simulink model "test_LQI_x"  (R2025b)
settings: Solver=VariableStepAuto  StartTime=0.0  StopTime=15  RelTol=1e-3
values from neighbouring files (symbols this model uses):
  Kd = 0.8 * K_aug(2)    [gains_LQI.m]
  Kd_theta = K_aug_theta(2)    [gains_LQI.m]
  Kd_x = 0.28    [gains_LQI.m]
  Ki = 0.8 * K_aug(3)    [gains_LQI.m]
  Ki_theta = K_aug_theta(3)    [gains_LQI.m]
  Kp = 0.8 * K_aug(1)    [gains_LQI.m]
  Kp_theta = K_aug_theta(1)    [gains_LQI.m]
  Kp_x = 0.23    [gains_LQI.m]
  tau = 1.2    [gains_LQI.m]
undefined symbols (not defined in the file or in its folder): DiscIntNeverNeededParam
libraries: simulink x2
settings Model: Creator=anoua  LastModifiedBy=anoua

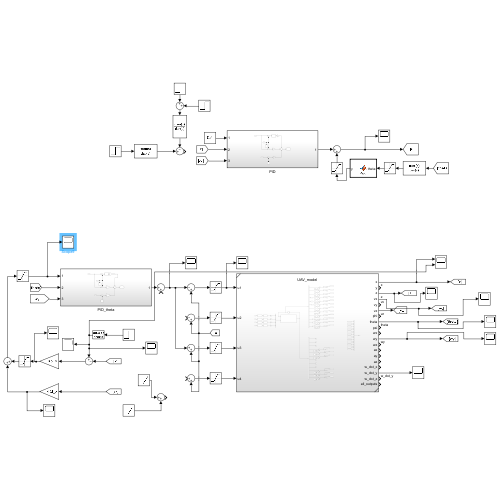
[thumbnail: Simulink's stored preview of the top-level diagram]
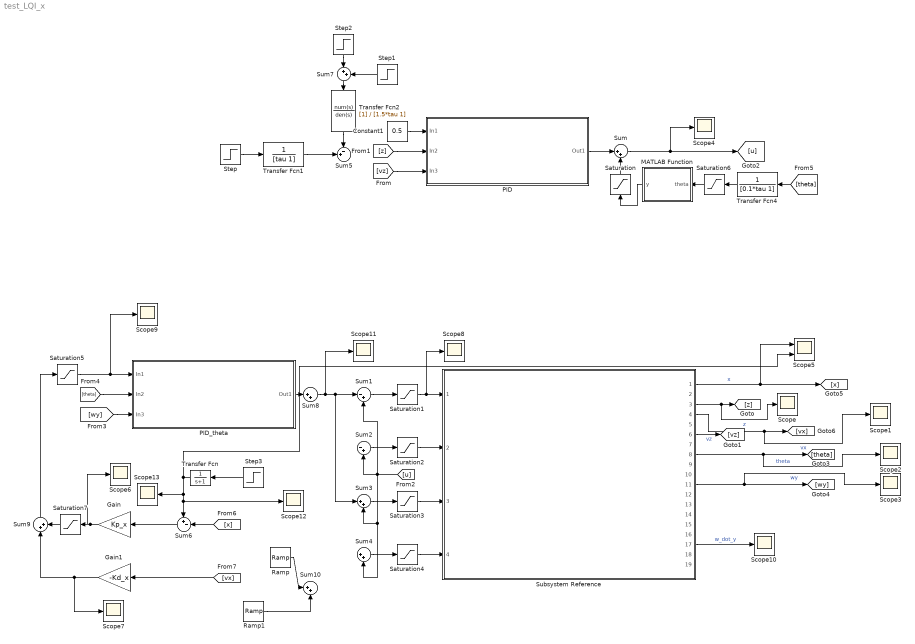
== system test_LQI_x ==
  Constant1 : Constant  Value=0.5
  Gain : Gain  Gain=Kp_x
  Gain1 : Gain  Gain=-Kd_x
  MATLAB Function : MATLAB Function  TreatAsAtomicUnit=on
  PID : Subsystem
  PID_theta : Subsystem
  Ramp : simulink/Sources/Ramp  slope=2  start=4  InitialOutput=0
  Ramp1 : simulink/Sources/Ramp  slope=-2  start=10  InitialOutput=0
  Saturation : Saturate  LowerLimit=0.3
  Saturation{1..4} (4 alike) : Saturate  UpperLimit=1  LowerLimit=-1
  Saturation5 : Saturate  UpperLimit=0.3  LowerLimit=-0.3  LinearizeAsGain=off
  Saturation6 : Saturate  UpperLimit=0.1  LowerLimit=0.1
  Saturation7 : Saturate  UpperLimit=1.5  LowerLimit=-1.5
  Scope{,1..4,6..13} (13 alike) : Scope
      Scope settings: ActiveDisplayYMinimum=-0.14718126227683057  ActiveDisplayYMaximum=0.70256454123979917
      Scope1 settings: ActiveDisplayYMinimum=-0.689477140233383  ActiveDisplayYMaximum=6.1817348155800982
      Scope10 settings: ActiveDisplayYMinimum=-8.1395929845312978  ActiveDisplayYMaximum=7.926459001284055  DataLoggingVariableName=ScopeData11
      Scope11 settings: ActiveDisplayYMinimum=-0.092583056017124382  ActiveDisplayYMaximum=0.10885517876194711  DataLoggingVariableName=ScopeData12
      Scope12 settings: ActiveDisplayYMinimum=-0.2209054413815989  ActiveDisplayYMaximum=0.24676727126462211  DataLoggingVariableName=ScopeData13
      Scope13 settings: ActiveDisplayYMinimum=-12.499998593310311  ActiveDisplayYMaximum=112.49998733979282  DataLoggingVariableName=ScopeData14
      Scope2 settings: ActiveDisplayYMinimum=-0.2429354271452315  ActiveDisplayYMaximum=0.30371803147303827  DataLoggingVariableName=ScopeData2
      Scope3 settings: ActiveDisplayYMinimum=-0.35804331506939135  ActiveDisplayYMaximum=2.2543304965066233  DataLoggingVariableName=ScopeData5
      Scope4 settings: ActiveDisplayYMinimum=-4.4218137268268194  ActiveDisplayYMaximum=39.350730126019634  DataLoggingVariableName=ScopeData4
      Scope6 settings: ActiveDisplayYMinimum=-3.5759205292689886  ActiveDisplayYMaximum=0.41468962885277622  DataLoggingVariableName=ScopeData7
      Scope7 settings: ActiveDisplayYMinimum=-1.5368936479557955  ActiveDisplayYMaximum=0.17077884596504492  DataLoggingVariableName=ScopeData8
      Scope8 settings: ActiveDisplayYMinimum=-0.17670639288242362  ActiveDisplayYMaximum=1.1307451547647138  DataLoggingVariableName=ScopeData9
      Scope9 settings: ActiveDisplayYMinimum=-0.28830610505236332  ActiveDisplayYMaximum=0.27997211142053136  DataLoggingVariableName=ScopeData10
  Scope5 : Scope  NumInputPorts=2
      settings: ActiveDisplayYMinimum=-0.6266529637915077  ActiveDisplayYMaximum=5.6296559852329642  DataLoggingVariableName=ScopeData6
  Step : Step  Time=0  After=0.5  SampleTime=0
  Step1 : Step  Time=16  After=0.70  SampleTime=0
  Step2 : Step  Time=22  After=0.05  SampleTime=0
  Step3 : Step  Time=4  After=5  SampleTime=0
  Subsystem Reference : Subsystem  ReferencedSubsystem=UAV_model
  Sum{,3..4,7..10} (7 alike) : Sum  Inputs=|++
  Sum1 : Sum  Inputs=|-+
  Sum2 : Sum  Inputs=|-+
  Sum5 : Sum  Inputs=-+|
  Sum6 : Sum  Inputs=+-|
  Transfer Fcn : TransferFcn  Denominator=[1 1]
  Transfer Fcn1 : TransferFcn  Denominator=[tau 1]
  Transfer Fcn2 : TransferFcn  Denominator=[1.5*tau 1]
  Transfer Fcn4 : TransferFcn  Denominator=[0.1*tau 1]
  wires:
  Subsystem Reference/3 -> Scope/1, [z]  "z"
  Sum/1 -> [u], Scope4/1
  [z] -> PID/2(In2)
  PID/1(Out1) -> Sum/1
  [vz] -> PID/3(In3)
  Sum2/1 -> Saturation2/1
  Sum7/1 -> Transfer Fcn2/1
  [u] -> Sum4/2, Sum3/2, Sum1/2, Sum2/2
  Saturation4/1 -> Subsystem Reference/4
  [theta] -> PID_theta/2(In2)
  Step1/1 -> Sum7/2
  [wy] -> PID_theta/3(In3)
  Step2/1 -> Sum7/1
  Transfer Fcn2/1 -> Sum5/1
  Saturation1/1 -> Scope8/1, Subsystem Reference/1
  Transfer Fcn1/1 -> Sum5/2
  Sum3/1 -> Saturation3/1
  Saturation3/1 -> Subsystem Reference/3
  Sum4/1 -> Saturation4/1
  Step/1 -> Transfer Fcn1/1
  Saturation2/1 -> Subsystem Reference/2
  Sum1/1 -> Saturation1/1
  Sum8/1 -> Scope11/1, Sum3/1, Sum1/1
  Subsystem Reference/11 -> Scope3/1, [wy]  "wy"
  Subsystem Reference/1 -> Scope5/1, [x]  "x"
  Constant1/1 -> PID/1(In1)
  MATLAB Function/1(y) -> Saturation/1
  [theta] -> Transfer Fcn4/1
  Transfer Fcn4/1 -> Saturation6/1
  Saturation/1 -> Sum/2
  Subsystem Reference/8 -> Scope2/1, [theta]  "theta"
  Subsystem Reference/17 -> Scope10/1  "w_dot_y"
  PID_theta/1(Out1) -> Sum8/1
  Subsystem Reference/4 -> Scope1/1, [vx]  "vx"
  [x] -> Sum6/2
  Sum6/1 -> Gain/1
  [vx] -> Gain1/1
  Gain/1 -> Scope6/1, Saturation7/1
  Gain1/1 -> Sum9/1, Scope7/1
  Sum9/1 -> Saturation5/1
  Saturation6/1 -> MATLAB Function/1(theta)
  Subsystem Reference/6 -> [vz]  "vz"
  Saturation5/1 -> Scope9/1, PID_theta/1(In1)
  Transfer Fcn/1 -> Scope13/1, Scope12/1, Sum6/1, Scope5/2
  Ramp/1 -> Sum10/1
  Ramp1/1 -> Sum10/2
  Step3/1 -> Transfer Fcn/1
  Saturation7/1 -> Sum9/2

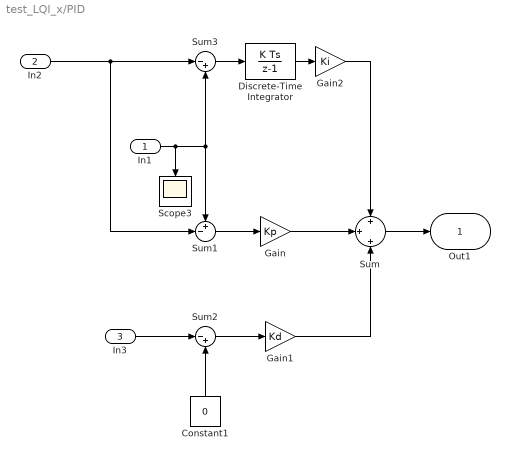
== system test_LQI_x/PID ==
  In1 : Inport
  In2 : Inport  Port=2
  In3 : Inport  Port=3
  Constant1 : Constant  Value=0
  Discrete-Time Integrator : DiscreteIntegrator  SampleTime=-1  LimitOutput=on  UpperSaturationLimit=1/Ki  LowerSaturationLimit=-1/Ki  ICPrevOutput=DiscIntNeverNeededParam  ICPrevScaledInput=DiscIntNeverNeededParam
  Gain : Gain  Gain=Kp
  Gain1 : Gain  Gain=Kd
  Gain2 : Gain  Gain=Ki
  Scope3 : Scope
      settings: ActiveDisplayYMinimum=-0.53484809981403014  ActiveDisplayYMaximum=1.6271171549271228  DataLoggingVariableName=ScopeData3
  Sum : Sum  Inputs=+|+|+
  Sum1 : Sum  Inputs=+-|
  Sum2 : Sum  Inputs=|-+
  Sum3 : Sum  Inputs=|-+
  Out1 : Outport
  wires:
  Gain2/1 -> Sum/1
  Gain/1 -> Sum/2
  Sum2/1 -> Gain1/1
  Gain1/1 -> Sum/3
  In1/1 -> Sum3/2, Sum1/1, Scope3/1
  Sum1/1 -> Gain/1
  Discrete-Time Integrator/1 -> Gain2/1
  Constant1/1 -> Sum2/2
  Sum3/1 -> Discrete-Time Integrator/1
  Sum/1 -> Out1/1
  In2/1 -> Sum1/2, Sum3/1
  In3/1 -> Sum2/1

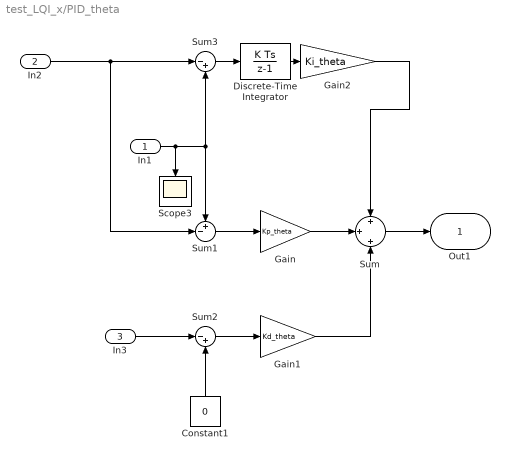
== system test_LQI_x/PID_theta ==
  In1 : Inport
  In2 : Inport  Port=2
  In3 : Inport  Port=3
  Constant1 : Constant  Value=0
  Discrete-Time Integrator : DiscreteIntegrator  SampleTime=-1  LimitOutput=on  UpperSaturationLimit=1/Ki_theta  LowerSaturationLimit=-1/Ki_theta  ICPrevOutput=DiscIntNeverNeededParam  ICPrevScaledInput=DiscIntNeverNeededParam
  Gain : Gain  Gain=Kp_theta
  Gain1 : Gain  Gain=Kd_theta
  Gain2 : Gain  Gain=Ki_theta
  Scope3 : Scope
      settings: ActiveDisplayYMinimum=-0.53484809981403014  ActiveDisplayYMaximum=1.6271171549271228  DataLoggingVariableName=ScopeData3
  Sum : Sum  Inputs=+|+|+
  Sum1 : Sum  Inputs=+-|
  Sum2 : Sum  Inputs=|-+
  Sum3 : Sum  Inputs=|-+
  Out1 : Outport
  wires:
  Gain2/1 -> Sum/1
  Gain/1 -> Sum/2
  Sum2/1 -> Gain1/1
  Gain1/1 -> Sum/3
  In1/1 -> Sum3/2, Sum1/1, Scope3/1
  Sum1/1 -> Gain/1
  Discrete-Time Integrator/1 -> Gain2/1
  Constant1/1 -> Sum2/2
  Sum3/1 -> Discrete-Time Integrator/1
  Sum/1 -> Out1/1
  In2/1 -> Sum1/2, Sum3/1
  In3/1 -> Sum2/1

== matlab function test_LQI_x/MATLAB Function ==
  data: theta input; y output
function y = fcn(theta)

y= 0.39/(cos(theta));
